simulink library "WECSim_Lib_Moorings"  (R2020b)
settings: Solver=VariableStepAuto  StartTime=0.0  StopTime=10.0  RelTol=1e-3
undefined symbols (not defined in the file or in its folder): mooring, simu, X, Y, Z
libraries: sm_lib x16, nesl_utility x6, $bdroot x6, WECSim_Lib_Body_Elements x3
settings Model: Creator=kmruehl  LastModifiedBy=jtgrasb

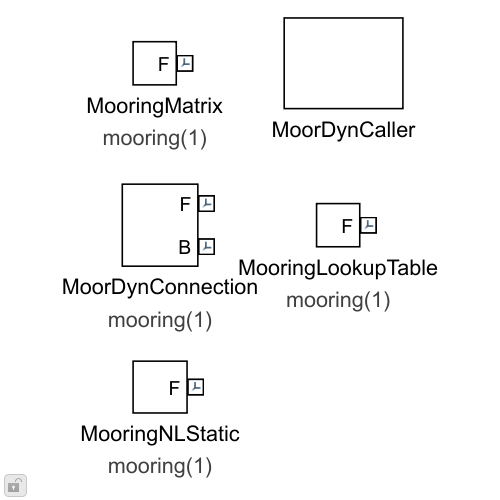
[thumbnail: Simulink's stored preview of the top-level diagram]
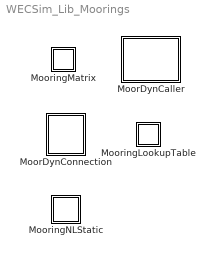
== system WECSim_Lib_Moorings ==
  MoorDynCaller : Subsystem  mask{simu=simu, mooring=mooring, InputFileText=Global Reference Frame option "Use Input File" is selected., numMoorDyn=0}
      mask prompts: simu "Simulation Class Name:"; mooring "Mooring Class Name:"; numMoorDyn "Number of MoorDyn Blocks"
      mask init:
      | if exist('mooring','var')
      |     h=[gcb '/Demux'];
      |     if str2num(get_param(h,'Outputs')) ~= simu.numMoorDyn
      |         % Delete old blocks
      |         fromBlocks = Simulink.findBlocks(gcb,'BlockType','From');
      |         gotoBlocks = Simulink.findBlocks(gcb,'BlockType','Goto');
      |         blocks = [fromBlocks;gotoBlocks];
      |         for ii=1:length(blocks)
      |             if ~contains(getfullname(blocks(ii)), 'Time')
      |                 line = get_param(blocks(ii),'LineHandles');
      |                 if line.Outport > 1
      |                     delete_line(line.Outport(1));
      |                 end
      |                 if line.Inport > 1
      |                     delete_line(line.Inport(1));
      |                 end
      |                 delete_block(blocks(ii))
      |             end
      |         end
      |         %% Set number of mux inputs and outputs
      |         h = [gcb '/muxDisp'];
      |         set_param(h,'Inputs',num2str(simu.numMoorDyn));
      |         h = [gcb '/muxVel'];
      |         set_param(h,'Inputs',num2str(simu.numMoorDyn));
      |         h = [gcb '/Demux'];
      |         set_param(h,'Outputs',num2str(simu.numMoorDyn));
      |         %% Add number of from and goto blocks according to MoorDyn connections
      |         for ii = 1:simu.numMoorDyn
      |             hDisp = add_block('simulink/Signal Routing/From',[gcb '/From'],'GotoTag',['moorDynDisp' num2str(ii)], 'MakeNameUnique', 'on');
      |             hVel = add_block('simulink/Signal Routing/From',[gcb '/From'],'GotoTag',['moorDynVel' num2str(ii)], 'MakeNameUnique', 'on');
      |             hForce = add_block('simulink/Signal Routing/Goto',[gcb '/Goto'],'GotoTag',['moorDynForce' num2str(ii)],'TagVisibility','global','MakeNameUnique', 'on');
      |             add_line(gcb,[get_param(hDisp,'Name') '/1'],[get_param([gcb '/muxDisp'],'Name') '/' num2str(ii)]);
      |             add_line(gcb,[get_param(hVel,'Name') '/1'],[get_param([gcb '/muxVel'],'Name') '/' num2str(ii)]);
      |             add_line(gcb,['Demux/' num2str(ii)],[get_param(hForce,'Name') '/1']);
      |         end
      |     end
      | end
      mask DialogControl InputFileGroup Prompt: Input File
      mask DialogControl CustomParameterGroup Prompt: Custom Parameters
      mask DialogControl mooringData Prompt: Mooring Data
      mask DialogControl simData Prompt: Simulation Data
  MoorDynConnection : Subsystem  mask(MoorDyn){mooring=mooring(1), InputFileText=Global Reference Frame option "Use Input File" is selected., MooringRef=0  0  0, moorDynLines=0}
      mask prompts: mooring "Mooring Name:"; MooringRef "Reference Location [m]:"; moorDynLines "Number of MoorDyn Lines:"
      mask help:
      | A mooring body that applies stiffness, damping and pretensions forces to the follower using a MoorDyn simulation. The response of the mooring body is relative to the global reference frame.
      |
      | The variable name input below must be 'mooring(i)' where i=1,2,...
      | mooring(i) must be defined in the input file with the following fields:
      |
      |     .name (required)
      |             String.
      |             Mooring name. Must comply with Matlab's variable naming rules.
      |     .location (optional)
      |             3x1 vector [x y z] in meters.
      |             Mooring location. Default = [0 0 0]
      |     .initial (optional)
      |             Struct
      |             Contains the initial position, angle and axis of the mooring body.
      |     .initial.displacement (optional)
      |             3x1 vector [x y z] in meters.
      |             Initial linear displacement from the ref position. Default = [0 0 0]
      |             This can can be set directly or with the setInitDisp() method.
      |     .initial.axis (optional)
      |             3x1 vector [x y z]
      |             Initial angular displacement axis. Default = [0 1 0]
      |             This can can be set directly or with the setInitDisp() method.
      |     .initial.angle (optional)
      |             Float.
      |             Initial angular displacement angle about axis in radians. Default = [0 0 0]
      |             This can can be set directly or with the setInitDisp() method.
      |     .moorDynLines (optional)
      |             Float.
      |             Number of lines for MoorDyn to use. Default = 0
      |     .moorDynNodes (optional)
      |             moorDynLines x 1 vector.
      |             Specifies the number of nodes per line in MoorDyn. Default = []
      mask init:
      | if exist('mooring','var')
      |     h=[gcb '/To Workspace'];
      |     responseName=['mooring' num2str(mooring.number) '_out'];
      |     set_param(h,'VariableName',responseName);
      |     % set from and goto block tags
      |     h=[gcb '/From'];
      |     set_param(h,'GotoTag',['moorDynForce' num2str(mooring.number)])
      |     h=[gcb '/Goto'];
      |     set_param(h,'GotoTag',['moorDynDisp' num2str(mooring.number)])
      |     h=[gcb '/Goto1'];
      |     set_param(h,'GotoTag',['moorDynVel' num2str(mooring.number)])
      | end
      settings: AttributesFormatString=%<mooring>
      mask Help:
      | A mooring body that applies stiffness, damping and pretensions forces to the follower using a MoorDyn simulation. The response of the mooring body is relative to the global reference frame.
      | 
      | The variable name input below must be 'mooring(i)' where i=1,2,...
      | mooring(i) must be defined in the input file with the following fields:
      | 
      |     .name (required)
      |             String.
      |             Mooring name. Must comply with Matlab's variable naming rules.
      |     .location (optional)
      |             3x1 vector [x y z] in meters.
      |             Mooring location. Default = [0 0 0]
      |     .initial (optional)
      |             Struct
      |             Contains the initial position, angle and axis of the mooring body.
      |     .initial.displacement (optional)
      |             3x1 vector [x y z] in meters.
      |             Initial linear displacement from the ref position. Default = [0 0 0]
      |             This can can be set directly or with the setInitDisp() method.
      |     .initial.axis (optional)
      |             3x1 vector [x y z]
      |             Initial angular displacement axis. Default = [0 1 0]
      |             This can can be set directly or with the setInitDisp() method.
      |     .initial.angle (optional)
      |             Float.
      |             Initial angular displacement angle about axis in radians. Default = [0 0 0]
      |             This can can be set directly or with the setInitDisp() method.
      |     .moorDynLines (optional)
      |             Float.
      |             Number of lines for MoorDyn to use. Default = 0
      |     .moorDynNodes (optional)
      |             moorDynLines x 1 vector.
      |             Specifies the number of nodes per line in MoorDyn. Default = []
      mask DialogControl InputFileGroup Prompt: Input File
      mask DialogControl CustomParameterGroup Prompt: Custom Parameters
      mask DialogControl mooringData Prompt: Mooring Data
  MooringLookupTable : Subsystem  mask{mooring=mooring(1)}
      mask prompts: mooring "Mooring Name:"
      mask init:
      | if exist('mooring','var')
      |     % toWorkSpace: outputs
      |     h=[gcb '/To Workspace'];
      |     responseName=['mooring' num2str(mooring.number) '_out'];
      |     set_param(h,'VariableName',responseName);
      | end
      settings: AttributesFormatString=%<mooring>
  MooringMatrix : Subsystem  mask(Mooring Matrix){mooring=mooring(1), InputFileText=Global Reference Frame option "Use Input File" is selected., loc=0 0 0, preTension=[0 0 0 0 0 0], stiffness={ '0', '0', '0', '0', '0', '0'; '0', '0', '0', '0', '0', '0'; '0', '0', '0', '0', '0', '0'; '0', '0', '0', '0', '0', '0'; '0', '0', '0', '0', '0', '0'; '0', '0', '0', '0', '0', '0' }, damping={ '0', '0', '0', '0', '0', '0'; '0', '0', '0', '0', '0', '0'; '0', '0', '0', '0', '0', '0'; '0', '0', '0', '0', '0', '0'; '0', '0', '0', '0', '0', '0'; '0', '0', '0', '0', '0', '0' }}
      mask prompts: mooring "Mooring Name:"; loc "Reference Location [m]:"; preTension "Pretension Force [N]:"; stiffness "Stiffness [N/m]:"; damping "Damping [N/m^2]:"
      mask help:
      | A mooring body that applies stiffness, damping and pretensions forces to the follower. The response of the mooring body is relative to the global reference frame.
      |
      | The variable name input below must be 'mooring(i)' where i=1,2,...
      | mooring(i) must be defined in the input file with the following fields:
      |
      |     .name (required)
      |             String.
      |             Mooring name. Must comply with Matlab's variable naming rules.
      |     .location (optional)
      |             3x1 vector [x y z] in meters.
      |             Mooring location. Default = [0 0 0]
      |     .initial (optional)
      |             Struct
      |             Contains the initial position, angle and axis of the mooring body.
      |     .initial.displacement (optional)
      |             3x1 vector [x y z] in meters.
      |             Initial linear displacement from the ref position. Default = [0 0 0]
      |             This can can be set directly or with the setInitDisp() method.
      |     .initial.axis (optional)
      |             3x1 vector [x y z]
      |             Initial angular displacement axis. Default = [0 1 0]
      |             This can can be set directly or with the setInitDisp() method.
      |     .initial.angle (optional)
      |             Float.
      |             Initial angular displacement angle about axis in radians. Default = [0 0 0]
      |             This can can be set directly or with the setInitDisp() method.
      |     .matrix (optional)
      |             Struct
      |             Contains the stiffness matrix, damping matrix and pretension of the mooring body.
      |     .matrix.stiffness (optional)
      |             6x6 vector.
      |             Mooring linear spring stiffness. Default = zeros(6)
      |     .matrix.damping (optional)
      |             6x6 vector.
      |             Mooring linear damping coefficient. Default = zeros(6)
      |     .matrix.preTension (optional)
      |             6x1 vector.
      |             Mooring preTension force. Default = [0 0 0 0 0 0]
      mask init:
      | if exist('mooring','var')
      |     % toWorkSpace: outputs
      |     h=[gcb '/To Workspace'];
      |     responseName=['mooring' num2str(mooring.number) '_out'];
      |     set_param(h,'VariableName',responseName);
      | end
      settings: AttributesFormatString=%<mooring>
      mask Help:
      | A mooring body that applies stiffness, damping and pretensions forces to the follower. The response of the mooring body is relative to the global reference frame.
      | 
      | The variable name input below must be 'mooring(i)' where i=1,2,...
      | mooring(i) must be defined in the input file with the following fields:
      | 
      |     .name (required)
      |             String.
      |             Mooring name. Must comply with Matlab's variable naming rules.
      |     .location (optional)
      |             3x1 vector [x y z] in meters.
      |             Mooring location. Default = [0 0 0]
      |     .initial (optional)
      |             Struct
      |             Contains the initial position, angle and axis of the mooring body.
      |     .initial.displacement (optional)
      |             3x1 vector [x y z] in meters.
      |             Initial linear displacement from the ref position. Default = [0 0 0]
      |             This can can be set directly or with the setInitDisp() method.
      |     .initial.axis (optional)
      |             3x1 vector [x y z]
      |             Initial angular displacement axis. Default = [0 1 0]
      |             This can can be set directly or with the setInitDisp() method.
      |     .initial.angle (optional)
      |             Float.
      |             Initial angular displacement angle about axis in radians. Default = [0 0 0]
      |             This can can be set directly or with the setInitDisp() method.
      |     .matrix (optional)
      |             Struct
      |             Contains the stiffness matrix, damping matrix and pretension of the mooring body.
      |     .matrix.stiffness (optional)
      |             6x6 vector.
      |             Mooring linear spring stiffness. Default = zeros(6)
      |     .matrix.damping (optional)
      |             6x6 vector.
      |             Mooring linear damping coefficient. Default = zeros(6)
      |     .matrix.preTension (optional)
      |             6x1 vector.
      |             Mooring preTension force. Default = [0 0 0 0 0 0]
      mask DialogControl InputFileGroup Prompt: Input File
      mask DialogControl CustomParameterGroup Prompt: Custom Parameters
      mask DialogControl matrix Prompt: Additional Parameters
  MooringNLStatic : Subsystem  mask(Mooring Matrix){mooring=mooring(1), nonlinearStaticData=mooring.nonlinearStaticData}
      mask prompts: mooring "Mooring Name:"; nonlinearStaticData "Mooring Data"
      mask help:
      | A mooring body that applies stiffness, damping and pretensions forces to the follower. The response of the mooring body is relative to the global reference frame.
      |
      | The variable name input below must be 'mooring(i)' where i=1,2,...
      | mooring(i) must be defined in the input file with the following fields:
      |
      |     .name (required)
      |             String.
      |             Mooring name. Must comply with Matlab's variable naming rules.
      |     .location (optional)
      |             3x1 vector [x y z] in meters.
      |             Mooring location. Default = [0 0 0]
      |     .initial (optional)
      |             Struct
      |             Contains the initial position, angle and axis of the mooring body.
      |     .initial.displacement (optional)
      |             3x1 vector [x y z] in meters.
      |             Initial linear displacement from the ref position. Default = [0 0 0]
      |             This can can be set directly or with the setInitDisp() method.
      |     .initial.axis (optional)
      |             3x1 vector [x y z]
      |             Initial angular displacement axis. Default = [0 1 0]
      |             This can can be set directly or with the setInitDisp() method.
      |     .initial.angle (optional)
      |             Float.
      |             Initial angular displacement angle about axis in radians. Default = [0 0 0]
      |             This can can be set directly or with the setInitDisp() method.
      |     .matrix (optional)
      |             Struct
      |             Contains the stiffness matrix, damping matrix and pretension of the mooring body.
      |     .matrix.stiffness (optional)
      |             6x6 vector.
      |             Mooring linear spring stiffness. Default = zeros(6)
      |     .matrix.damping (optional)
      |             6x6 vector.
      |             Mooring linear damping coefficient. Default = zeros(6)
      |     .matrix.preTension (optional)
      |             6x1 vector.
      |             Mooring preTension force. Default = [0 0 0 0 0 0]
      mask init:
      | if exist('mooring','var')
      |     % toWorkSpace: outputs
      |     h=[gcb '/To Workspace'];
      |     responseName=['mooring' num2str(mooring.number) '_out'];
      |     set_param(h,'VariableName',responseName);
      | end
      settings: AttributesFormatString=%<mooring>
      mask Help:
      | A mooring body that applies stiffness, damping and pretensions forces to the follower. The response of the mooring body is relative to the global reference frame.
      | 
      | The variable name input below must be 'mooring(i)' where i=1,2,...
      | mooring(i) must be defined in the input file with the following fields:
      | 
      |     .name (required)
      |             String.
      |             Mooring name. Must comply with Matlab's variable naming rules.
      |     .location (optional)
      |             3x1 vector [x y z] in meters.
      |             Mooring location. Default = [0 0 0]
      |     .initial (optional)
      |             Struct
      |             Contains the initial position, angle and axis of the mooring body.
      |     .initial.displacement (optional)
      |             3x1 vector [x y z] in meters.
      |             Initial linear displacement from the ref position. Default = [0 0 0]
      |             This can can be set directly or with the setInitDisp() method.
      |     .initial.axis (optional)
      |             3x1 vector [x y z]
      |             Initial angular displacement axis. Default = [0 1 0]
      |             This can can be set directly or with the setInitDisp() method.
      |     .initial.angle (optional)
      |             Float.
      |             Initial angular displacement angle about axis in radians. Default = [0 0 0]
      |             This can can be set directly or with the setInitDisp() method.
      |     .matrix (optional)
      |             Struct
      |             Contains the stiffness matrix, damping matrix and pretension of the mooring body.
      |     .matrix.stiffness (optional)
      |             6x6 vector.
      |             Mooring linear spring stiffness. Default = zeros(6)
      |     .matrix.damping (optional)
      |             6x6 vector.
      |             Mooring linear damping coefficient. Default = zeros(6)
      |     .matrix.preTension (optional)
      |             6x1 vector.
      |             Mooring preTension force. Default = [0 0 0 0 0 0]

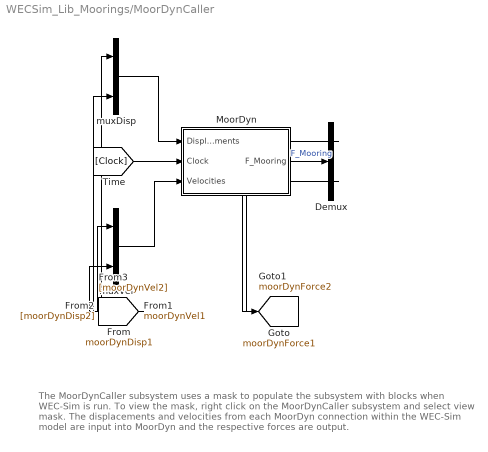
== system WECSim_Lib_Moorings/MoorDynCaller ==
  note: The MoorDynCaller subsystem uses a mask to populate the subsystem with blocks when WEC-Sim is run. To view the mask, right click on the MoorDynCaller subsystem and select view mask. The displacements and velocities from each MoorDyn connection within the WEC-Sim model are input into MoorDyn and the respective forces are output.
  Demux : Demux  Outputs=2
  MoorDyn : Subsystem  VariantControl=sv_moorDyn
  muxDisp : Mux  Inputs=2
  muxVel : Mux  Inputs=2
  tag scope: moorDynForce1=global, moorDynForce2=global
  wires:
  MoorDyn/1(F_Mooring) -> Demux/1  "F_Mooring"
  muxVel/1 -> MoorDyn/3(Velocities)
  muxDisp/1 -> MoorDyn/1(Displacements)
  [Clock] -> MoorDyn/2(Clock)
  [moorDynDisp1] -> muxDisp/1
  [moorDynVel1] -> muxVel/1
  Demux/1 -> [moorDynForce1]
  [moorDynDisp2] -> muxDisp/2
  [moorDynVel2] -> muxVel/2
  Demux/2 -> [moorDynForce2]

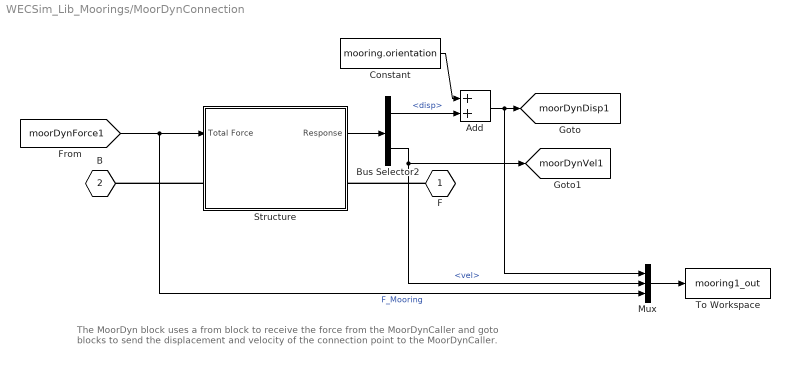
== system WECSim_Lib_Moorings/MoorDynConnection ==
  note: The MoorDyn block uses a from block to receive the force from the MoorDynCaller and goto blocks to send the displacement and velocity of the connection point to the MoorDynCaller.
  Add : Sum
  Bus Selector2 : BusSelector  OutputSignals=disp,vel
  Constant : Constant  Value=mooring.orientation
  Mux : Mux  Inputs=3
  Structure : Subsystem
  To Workspace : ToWorkspace  VariableName=mooring1_out  SaveFormat=Structure With Time  SampleTime=simu.dtOut
  F : PMIOPort  Side=Left
  B : PMIOPort  Port=2  Side=Left
  tag scope: moorDynDisp1=global, moorDynVel1=global
  wires:
  Add/1 -> [moorDynDisp1], Mux/1
  Constant/1 -> Add/1
  Bus Selector2/2 -> Mux/2, [moorDynVel1]  "<vel>"
  Mux/1 -> To Workspace/1
  Bus Selector2/1 -> Add/2  "<disp>"
  [moorDynForce1] -> Structure/1(Total Force), Mux/3  "F_Mooring"
  Structure/1(Response) -> Bus Selector2/1
  connections:
  F/RConn1 -- Structure/RConn1
  Structure/LConn1 -- B/RConn1

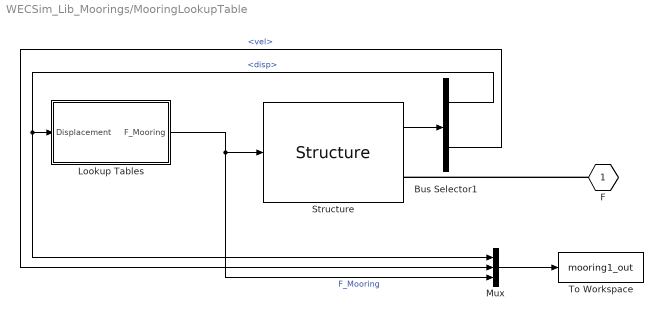
== system WECSim_Lib_Moorings/MooringLookupTable ==
  Bus Selector1 : BusSelector  OutputSignals=disp,vel
  Lookup Tables : Subsystem
  Mux : Mux  Inputs=3
  Structure : $bdroot/MooringMatrix/Structure  SystemSampleTime=-1  VariantActivationTime=update diagram  Latency=0  AutoFrameSizeCalculation=off
      link override Body Properties: GraphicType=None
  To Workspace : ToWorkspace  VariableName=mooring1_out  SaveFormat=Structure With Time  SampleTime=simu.dtOut
  F : PMIOPort  Side=Left
  wires:
  Mux/1 -> To Workspace/1
  Bus Selector1/2 -> Mux/2  "<vel>"
  Bus Selector1/1 -> Mux/1, Lookup Tables/1(Displacement)  "<disp>"
  Lookup Tables/1(F_Mooring) -> Mux/3, Structure/1  "F_Mooring"
  Structure/1 -> Bus Selector1/1
  connections:
  F/RConn1 -- Structure/RConn1

== system WECSim_Lib_Moorings/MooringMatrix ==
  Bus Selector2 : BusSelector  OutputSignals=disp,vel
  Mooring Matrix : Subsystem  VariantControl=sv_mooringMatrix
  Mux : Mux  Inputs=3
  Structure : Subsystem
  To Workspace : ToWorkspace  VariableName=mooring1_out  SaveFormat=Structure With Time  SampleTime=simu.dtOut
  F : PMIOPort  Side=Left
  wires:
  Structure/1(Response) -> Bus Selector2/1
  Mooring Matrix/1(F_Mooring) -> Mux/3, Structure/1(Total Force)  "F_Mooring"
  Bus Selector2/1 -> Mux/1, Mooring Matrix/1(Displacement)  "<disp>"
  Bus Selector2/2 -> Mux/2, Mooring Matrix/2(Velocity)  "<vel>"
  Mux/1 -> To Workspace/1
  connections:
  F/RConn1 -- Structure/RConn1

== system WECSim_Lib_Moorings/MooringNLStatic ==
  Bus Selector2 : BusSelector  OutputSignals=disp,vel
  Mooring Matrix : Subsystem  VariantControl=sv_mooringMatrix
  Mux : Mux  Inputs=3
  Structure : Subsystem
  To Workspace : ToWorkspace  VariableName=mooring1_out  SaveFormat=Structure With Time  SampleTime=simu.dtOut
  F : PMIOPort  Side=Left
  wires:
  Mux/1 -> To Workspace/1
  Bus Selector2/2 -> Mux/2  "<vel>"
  Bus Selector2/1 -> Mooring Matrix/1(Displacement), Mux/1  "<disp>"
  Mooring Matrix/1(F_Mooring) -> Structure/1(Total Force), Mux/3  "F_Mooring"
  Structure/1(Response) -> Bus Selector2/1
  connections:
  F/RConn1 -- Structure/RConn1

== system WECSim_Lib_Moorings/MoorDynCaller/MoorDyn ==
  Displacements : Inport
  Clock : Inport  Port=2
  Velocities : Inport  Port=3
  MoorDyn : Subsystem
  F_Mooring : Outport
  wires:
  MoorDyn/1(Flines) -> F_Mooring/1
  Clock/1 -> MoorDyn/2(Clock)
  Displacements/1 -> MoorDyn/3(Displacements)
  Velocities/1 -> MoorDyn/1(Velocities)

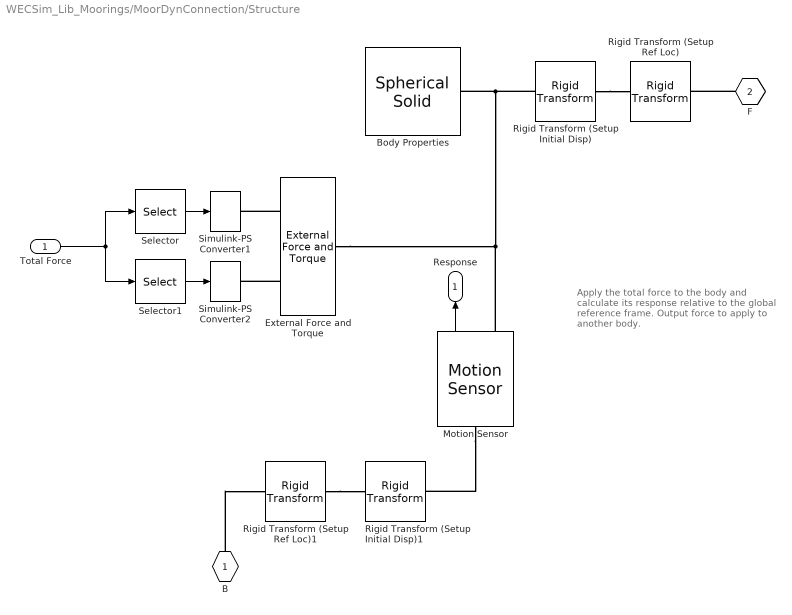
== system WECSim_Lib_Moorings/MoorDynConnection/Structure ==
  note: Apply the total force to the body and calculate its response relative to the global reference frame.
      |
      | Output force to apply to another body.
  Total Force : Inport
  Body Properties : sm_lib/Body Elements/Spherical Solid  GraphicAmbientColor=[0.15 0.15 0.15 1.0]  BasedOnType=Density  CenterOfMass=[0 0 0]  CenterOfMassUnits=m  GraphicDiffuseColor=[0 1 0]  Density=1000  DensityUnits=kg/(m^3)  DoExposeReferenceFrame=on  GraphicEmissiveColor=[0.0 0.0 0.0 1.0]  ExportEntireGeometry=off  SerializedExposedGeometries=<ExposedGeometries/>  SerializedFrames=<Frames/>  MarkerShape=Sphere  MarkerSize=10  GraphicType=None  InertiaType=Custom  Mass=0  MassUnits=kg  MomentsOfInertia=[0 0 0]  MomentsOfInertiaUnits=kg*m^2  GraphicOpacity=1  ProductsOfInertia=[0 0 0]  ProductsOfInertiaUnits=kg*m^2  GraphicShininess=75  GraphicSpecularColor=[0.5 0.5 0.5 1.0]  SphereRadius=1  SphereRadiusUnits=m  GraphicVisPropType=SimpleVisualProperties
  External Force and Torque : sm_lib/Forces and Torques/External Force and Torque  ForceResolutionFrame=World  EnableForceX=off  EnableForceY=off  EnableForceZ=off  EnableForce=on  TorqueResolutionFrame=World  EnableTorqueX=off  EnableTorqueY=off  EnableTorqueZ=off  EnableTorque=on
  Motion Sensor : WECSim_Lib_Body_Elements/Rigid Body/Hydrodynamic Body/Structure/Motion Sensor  SystemSampleTime=-1  VariantActivationTime=update diagram  Latency=0  AutoFrameSizeCalculation=off
  Rigid Transform (Setup Initial Disp) : sm_lib/Frames and Transforms/Rigid Transform  TranslationMethod=Cartesian  TranslationStandardOffset=0  TranslationStandardOffsetUnits=m  TranslationStandardAxis=+Z  TranslationCartesianOffset=mooring.initial.displacement  TranslationCartesianOffsetUnits=m  TranslationROffset=0  TranslationROffsetUnits=m  TranslationZOffset=0  TranslationZOffsetUnits=m  TranslationThetaOffset=0  TranslationThetaOffsetUnits=deg  RotationMethod=ArbitraryAxis  RotationAngleUnits=rad  RotationStandardAxis=+Y  RotationAngle=mooring.initial.angle  RotationArbitraryAxis=mooring.initial.axis  FollAlignAxisA=+X  BaseAlignAxisA=+Y  FollAlignAxisB=+Y  BaseAlignAxisB=+Z  RotationSequenceAxes=FollowerAxes  RotationSequence=XYX  RotationSequenceAngles=[0 0 0]  RotationSequenceAnglesUnits=deg  RotationMatrix=[1 0 0; 0 1 0; 0 0 1]  Quaternion=[1 0 0 0]
  Rigid Transform (Setup Initial Disp)1 : sm_lib/Frames and Transforms/Rigid Transform  TranslationMethod=Cartesian  TranslationStandardOffset=0  TranslationStandardOffsetUnits=m  TranslationStandardAxis=+Z  TranslationCartesianOffset=mooring.initial.displacement  TranslationCartesianOffsetUnits=m  TranslationROffset=0  TranslationROffsetUnits=m  TranslationZOffset=0  TranslationZOffsetUnits=m  TranslationThetaOffset=0  TranslationThetaOffsetUnits=deg  RotationMethod=ArbitraryAxis  RotationAngleUnits=rad  RotationStandardAxis=+Y  RotationAngle=mooring.initial.angle  RotationArbitraryAxis=mooring.initial.axis  FollAlignAxisA=+X  BaseAlignAxisA=+Y  FollAlignAxisB=+Y  BaseAlignAxisB=+Z  RotationSequenceAxes=FollowerAxes  RotationSequence=XYX  RotationSequenceAngles=[0 0 0]  RotationSequenceAnglesUnits=deg  RotationMatrix=[1 0 0; 0 1 0; 0 0 1]  Quaternion=[1 0 0 0]
  Rigid Transform (Setup Ref Loc) : sm_lib/Frames and Transforms/Rigid Transform  TranslationMethod=Cartesian  TranslationStandardOffset=0  TranslationStandardOffsetUnits=m  TranslationStandardAxis=+Z  TranslationCartesianOffset=mooring.location  TranslationCartesianOffsetUnits=m  TranslationROffset=0  TranslationROffsetUnits=m  TranslationZOffset=0  TranslationZOffsetUnits=m  TranslationThetaOffset=0  TranslationThetaOffsetUnits=deg  RotationMethod=None  RotationAngleUnits=rad  RotationStandardAxis=+Y  RotationAngle=0.05  RotationArbitraryAxis=[0.57735026918962584 0.57735026918962584 0.57735026918962584]  FollAlignAxisA=+X  BaseAlignAxisA=+Y  FollAlignAxisB=+Y  BaseAlignAxisB=+Z  RotationSequenceAxes=FollowerAxes  RotationSequence=XYX  RotationSequenceAngles=[0 0 0]  RotationSequenceAnglesUnits=deg  RotationMatrix=[1 0 0; 0 1 0; 0 0 1]  Quaternion=[1 0 0 0]
  Rigid Transform (Setup Ref Loc)1 : sm_lib/Frames and Transforms/Rigid Transform  TranslationMethod=Cartesian  TranslationStandardOffset=0  TranslationStandardOffsetUnits=m  TranslationStandardAxis=+Z  TranslationCartesianOffset=mooring.location  TranslationCartesianOffsetUnits=m  TranslationROffset=0  TranslationROffsetUnits=m  TranslationZOffset=0  TranslationZOffsetUnits=m  TranslationThetaOffset=0  TranslationThetaOffsetUnits=deg  RotationMethod=None  RotationAngleUnits=rad  RotationStandardAxis=+Y  RotationAngle=0.05  RotationArbitraryAxis=[0.57735026918962584 0.57735026918962584 0.57735026918962584]  FollAlignAxisA=+X  BaseAlignAxisA=+Y  FollAlignAxisB=+Y  BaseAlignAxisB=+Z  RotationSequenceAxes=FollowerAxes  RotationSequence=XYX  RotationSequenceAngles=[0 0 0]  RotationSequenceAnglesUnits=deg  RotationMatrix=[1 0 0; 0 1 0; 0 0 1]  Quaternion=[1 0 0 0]
  Selector : Selector  InputPortWidth=6  IndexOptions=Index vector (dialog)  Indices=[1:3]  OutputSizes=1
  Selector1 : Selector  InputPortWidth=6  IndexOptions=Index vector (dialog)  Indices=[4:6]  OutputSizes=1
  Simulink-PS Converter1 : nesl_utility/Simulink-PS Converter  PhysicalDomain=network_engine_domain  SubClassName=ps_input  LeftPortType=input  RightPortType=output  PseudoPeriodic=off  Frequencies=[]  NoiseDistribution=none  NoiseParameters=[]  Unit=1  AffineConversion=off  FilteringAndDerivatives=zero  SimscapeFilterOrder=1  InputFilterTimeConstant=0.001  UdotUserProvided=1
  Simulink-PS Converter2 : nesl_utility/Simulink-PS Converter  PhysicalDomain=network_engine_domain  SubClassName=ps_input  LeftPortType=input  RightPortType=output  PseudoPeriodic=off  Frequencies=[]  NoiseDistribution=none  NoiseParameters=[]  Unit=1  AffineConversion=off  FilteringAndDerivatives=zero  SimscapeFilterOrder=1  InputFilterTimeConstant=0.001  UdotUserProvided=1
  B : PMIOPort  Side=Left
  F : PMIOPort  Port=2  Side=Right
  Response : Outport
  wires:
  Total Force/1 -> Selector1/1, Selector/1
  Selector/1 -> Simulink-PS Converter1/1
  Selector1/1 -> Simulink-PS Converter2/1
  Motion Sensor/1 -> Response/1
  connections:
  Rigid Transform (Setup Ref Loc)1/RConn1 -- Rigid Transform (Setup Initial Disp)1/LConn1
  Motion Sensor/LConn1 -- Rigid Transform (Setup Initial Disp)1/RConn1
  External Force and Torque/LConn1 -- Simulink-PS Converter1/RConn1
  External Force and Torque/LConn2 -- Simulink-PS Converter2/RConn1
  Rigid Transform (Setup Initial Disp)/RConn1 -- Body Properties/RConn1 -- Motion Sensor/RConn1 -- External Force and Torque/RConn1
  F/RConn1 -- Rigid Transform (Setup Ref Loc)/LConn1
  Rigid Transform (Setup Initial Disp)/LConn1 -- Rigid Transform (Setup Ref Loc)/RConn1
  B/RConn1 -- Rigid Transform (Setup Ref Loc)1/LConn1

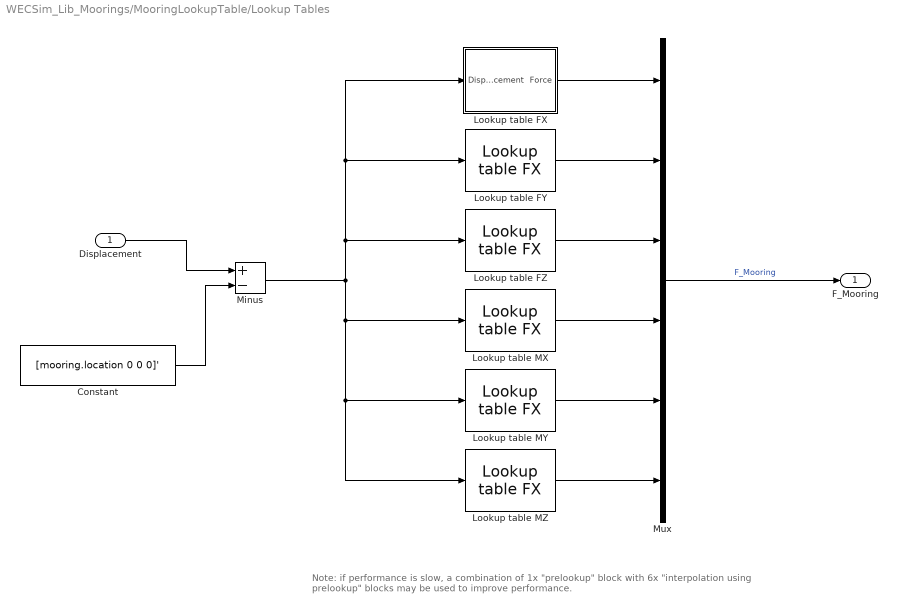
== system WECSim_Lib_Moorings/MooringLookupTable/Lookup Tables ==
  note: Note: if performance is slow, a combination of 1x "prelookup" block with 6x "interpolation using prelookup" blocks may be used to improve performance.
  Displacement : Inport
  Constant : Constant  Value=[mooring.location 0 0 0]'
  Lookup table FX : Subsystem  mask{forceComponent=mooring.lookupTable.FX}
      mask prompts: forceComponent "Force component:"
  Lookup table FY : $bdroot/MooringLookupTable/Lookup Tables/Lookup table FX  forceComponent=mooring.lookupTable.FY
  Lookup table FZ : $bdroot/MooringLookupTable/Lookup Tables/Lookup table FX  forceComponent=mooring.lookupTable.FZ
  Lookup table MX : $bdroot/MooringLookupTable/Lookup Tables/Lookup table FX  forceComponent=mooring.lookupTable.MX
  Lookup table MY : $bdroot/MooringLookupTable/Lookup Tables/Lookup table FX  forceComponent=mooring.lookupTable.MY
  Lookup table MZ : $bdroot/MooringLookupTable/Lookup Tables/Lookup table FX  forceComponent=mooring.lookupTable.MZ
  Minus : Sum  Inputs=+-
  Mux : Mux  Inputs=6
  F_Mooring : Outport
  wires:
  Minus/1 -> Lookup table MX/1, Lookup table MZ/1, Lookup table MY/1, Lookup table FY/1, Lookup table FX/1(Displacement), Lookup table FZ/1
  Lookup table MZ/1 -> Mux/6
  Lookup table MY/1 -> Mux/5
  Lookup table MX/1 -> Mux/4
  Lookup table FZ/1 -> Mux/3
  Lookup table FY/1 -> Mux/2
  Lookup table FX/1(Force) -> Mux/1
  Mux/1 -> F_Mooring/1  "F_Mooring"
  Displacement/1 -> Minus/1
  Constant/1 -> Minus/2

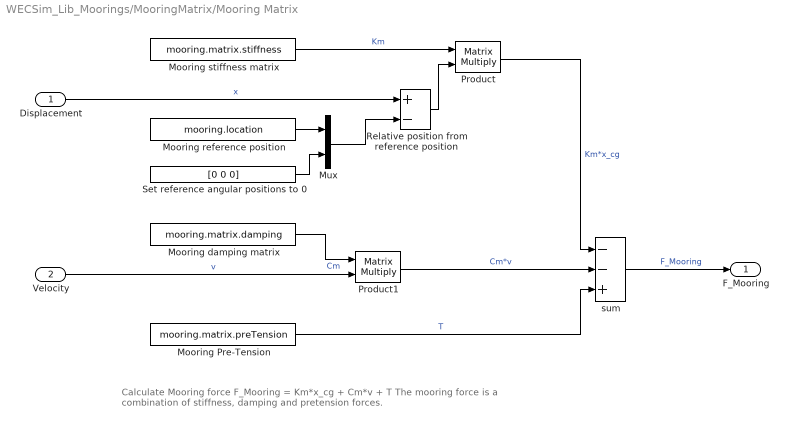
== system WECSim_Lib_Moorings/MooringMatrix/Mooring Matrix ==
  note: Calculate Mooring force
      |
      | F_Mooring = Km*x_cg + Cm*v + T
      | The mooring force is a combination of stiffness, damping and pretension forces.
  Displacement : Inport
  Velocity : Inport  Port=2
  Mooring Pre-Tension : Constant  Value=mooring.matrix.preTension
  Mooring damping matrix : Constant  Value=mooring.matrix.damping
  Mooring reference position : Constant  Value=mooring.location
  Mooring stiffness matrix : Constant  Value=mooring.matrix.stiffness
  Mux : Mux  Inputs=2
  Product : Product  Multiplication=Matrix(*)
  Product1 : Product  Multiplication=Matrix(*)
  Relative position from reference position : Sum  Inputs=+-
  Set reference angular positions to 0 : Constant  Value=[0 0 0]
  sum : Sum  Inputs=--+
  F_Mooring : Outport
  wires:
  Product/1 -> sum/1  "Km*x_cg"
  Product1/1 -> sum/2  "Cm*v"
  sum/1 -> F_Mooring/1  "F_Mooring"
  Mooring Pre-Tension/1 -> sum/3  "T"
  Mooring stiffness matrix/1 -> Product/1  "Km"
  Velocity/1 -> Product1/2  "v"
  Mooring damping matrix/1 -> Product1/1  "Cm"
  Displacement/1 -> Relative position from reference position/1  "x"
  Mooring reference position/1 -> Mux/1
  Set reference angular positions to 0/1 -> Mux/2
  Mux/1 -> Relative position from reference position/2
  Relative position from reference position/1 -> Product/2

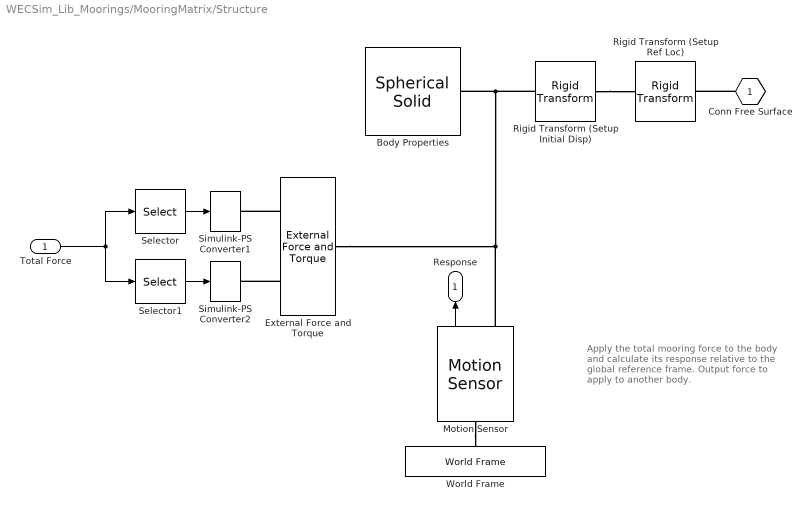
== system WECSim_Lib_Moorings/MooringMatrix/Structure ==
  note: Apply the total mooring force to the body and calculate its response relative to the global reference frame.
      |
      | Output force to apply to another body.
  Total Force : Inport
  Body Properties : sm_lib/Body Elements/Spherical Solid  GraphicAmbientColor=[0.15 0.15 0.15 1.0]  BasedOnType=Density  CenterOfMass=[0 0 0]  CenterOfMassUnits=m  GraphicDiffuseColor=[0.4 0.4 0.4]  Density=1000  DensityUnits=kg/(m^3)  DoExposeReferenceFrame=on  GraphicEmissiveColor=[0.0 0.0 0.0 1.0]  ExportEntireGeometry=off  SerializedExposedGeometries=<ExposedGeometries/>  SerializedFrames=<Frames/>  MarkerShape=Sphere  MarkerSize=10  GraphicType=Marker  InertiaType=Custom  Mass=0  MassUnits=kg  MomentsOfInertia=[0 0 0]  MomentsOfInertiaUnits=kg*m^2  GraphicOpacity=1  ProductsOfInertia=[0 0 0]  ProductsOfInertiaUnits=kg*m^2  GraphicShininess=75  GraphicSpecularColor=[0.5 0.5 0.5 1.0]  SphereRadius=5  SphereRadiusUnits=m  GraphicVisPropType=SimpleVisualProperties
  External Force and Torque : sm_lib/Forces and Torques/External Force and Torque  ForceResolutionFrame=World  EnableForceX=off  EnableForceY=off  EnableForceZ=off  EnableForce=on  TorqueResolutionFrame=World  EnableTorqueX=off  EnableTorqueY=off  EnableTorqueZ=off  EnableTorque=on
  Motion Sensor : WECSim_Lib_Body_Elements/Rigid Body/Hydrodynamic Body/Structure/Motion Sensor  SystemSampleTime=-1  VariantActivationTime=update diagram  Latency=0  AutoFrameSizeCalculation=off
  Rigid Transform (Setup Initial Disp) : sm_lib/Frames and Transforms/Rigid Transform  TranslationMethod=Cartesian  TranslationStandardOffset=0  TranslationStandardOffsetUnits=m  TranslationStandardAxis=+Z  TranslationCartesianOffset=mooring.initial.displacement  TranslationCartesianOffsetUnits=m  TranslationROffset=0  TranslationROffsetUnits=m  TranslationZOffset=0  TranslationZOffsetUnits=m  TranslationThetaOffset=0  TranslationThetaOffsetUnits=deg  RotationMethod=ArbitraryAxis  RotationAngleUnits=rad  RotationStandardAxis=+Y  RotationAngle=mooring.initial.angle  RotationArbitraryAxis=mooring.initial.axis  FollAlignAxisA=+X  BaseAlignAxisA=+Y  FollAlignAxisB=+Y  BaseAlignAxisB=+Z  RotationSequenceAxes=FollowerAxes  RotationSequence=XYX  RotationSequenceAngles=[0 0 0]  RotationSequenceAnglesUnits=deg  RotationMatrix=[1 0 0; 0 1 0; 0 0 1]  Quaternion=[1 0 0 0]
  Rigid Transform (Setup Ref Loc) : sm_lib/Frames and Transforms/Rigid Transform  TranslationMethod=Cartesian  TranslationStandardOffset=0  TranslationStandardOffsetUnits=m  TranslationStandardAxis=+Z  TranslationCartesianOffset=mooring.location  TranslationCartesianOffsetUnits=m  TranslationROffset=0  TranslationROffsetUnits=m  TranslationZOffset=0  TranslationZOffsetUnits=m  TranslationThetaOffset=0  TranslationThetaOffsetUnits=deg  RotationMethod=None  RotationAngleUnits=rad  RotationStandardAxis=+Y  RotationAngle=0.05  RotationArbitraryAxis=[0.57735026918962584 0.57735026918962584 0.57735026918962584]  FollAlignAxisA=+X  BaseAlignAxisA=+Y  FollAlignAxisB=+Y  BaseAlignAxisB=+Z  RotationSequenceAxes=FollowerAxes  RotationSequence=XYX  RotationSequenceAngles=[0 0 0]  RotationSequenceAnglesUnits=deg  RotationMatrix=[1 0 0; 0 1 0; 0 0 1]  Quaternion=[1 0 0 0]
  Selector : Selector  InputPortWidth=6  IndexOptions=Index vector (dialog)  Indices=[1:3]  OutputSizes=1
  Selector1 : Selector  InputPortWidth=6  IndexOptions=Index vector (dialog)  Indices=[4:6]  OutputSizes=1
  Simulink-PS Converter1 : nesl_utility/Simulink-PS Converter  PhysicalDomain=network_engine_domain  SubClassName=ps_input  LeftPortType=input  RightPortType=output  PseudoPeriodic=off  Frequencies=[]  NoiseDistribution=none  NoiseParameters=[]  Unit=1  AffineConversion=off  FilteringAndDerivatives=zero  SimscapeFilterOrder=1  InputFilterTimeConstant=0.001  UdotUserProvided=1
  Simulink-PS Converter2 : nesl_utility/Simulink-PS Converter  PhysicalDomain=network_engine_domain  SubClassName=ps_input  LeftPortType=input  RightPortType=output  PseudoPeriodic=off  Frequencies=[]  NoiseDistribution=none  NoiseParameters=[]  Unit=1  AffineConversion=off  FilteringAndDerivatives=zero  SimscapeFilterOrder=1  InputFilterTimeConstant=0.001  UdotUserProvided=1
  World Frame : sm_lib/Frames and Transforms/World Frame
  Conn Free Surface : PMIOPort  Side=Right
  Response : Outport
  wires:
  Total Force/1 -> Selector1/1, Selector/1
  Selector/1 -> Simulink-PS Converter1/1
  Selector1/1 -> Simulink-PS Converter2/1
  Motion Sensor/1 -> Response/1
  connections:
  External Force and Torque/LConn1 -- Simulink-PS Converter1/RConn1
  External Force and Torque/LConn2 -- Simulink-PS Converter2/RConn1
  Rigid Transform (Setup Initial Disp)/RConn1 -- Body Properties/RConn1 -- Motion Sensor/RConn1 -- External Force and Torque/RConn1
  Conn Free Surface/RConn1 -- Rigid Transform (Setup Ref Loc)/LConn1
  Rigid Transform (Setup Initial Disp)/LConn1 -- Rigid Transform (Setup Ref Loc)/RConn1
  Motion Sensor/LConn1 -- World Frame/RConn1

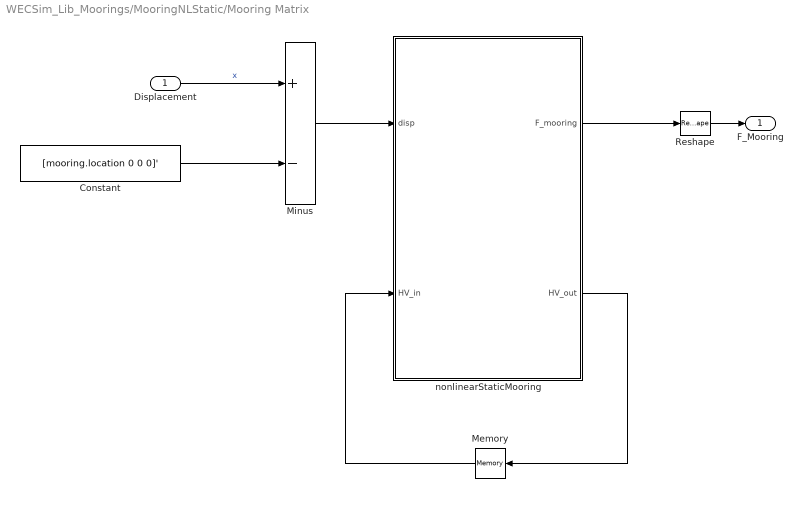
== system WECSim_Lib_Moorings/MooringNLStatic/Mooring Matrix ==
  Displacement : Inport
  Constant : Constant  Value=[mooring.location 0 0 0]'
  Memory : Memory  InitialCondition=nonlinearStaticData.HV0
  Minus : Sum  Inputs=+-
  Reshape : Reshape
  nonlinearStaticMooring : MATLAB Function  TreatAsAtomicUnit=on
  F_Mooring : Outport
  wires:
  Reshape/1 -> F_Mooring/1
  Displacement/1 -> Minus/1  "x"
  Constant/1 -> Minus/2
  nonlinearStaticMooring/1(F_mooring) -> Reshape/1
  nonlinearStaticMooring/2(HV_out) -> Memory/1
  Memory/1 -> nonlinearStaticMooring/2(HV_in)
  Minus/1 -> nonlinearStaticMooring/1(disp)

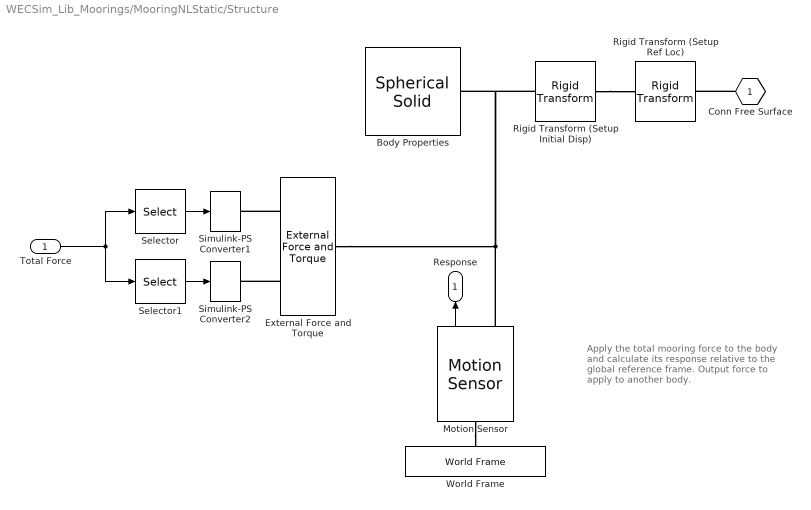
== system WECSim_Lib_Moorings/MooringNLStatic/Structure ==
  note: Apply the total mooring force to the body and calculate its response relative to the global reference frame.
      |
      | Output force to apply to another body.
  Total Force : Inport
  Body Properties : sm_lib/Body Elements/Spherical Solid  GraphicAmbientColor=[0.15 0.15 0.15 1.0]  BasedOnType=Density  CenterOfMass=[0 0 0]  CenterOfMassUnits=m  GraphicDiffuseColor=[0 1 0]  Density=1000  DensityUnits=kg/(m^3)  DoExposeReferenceFrame=on  GraphicEmissiveColor=[0.0 0.0 0.0 1.0]  ExportEntireGeometry=off  SerializedExposedGeometries=<ExposedGeometries/>  SerializedFrames=<Frames/>  MarkerShape=Sphere  MarkerSize=10  GraphicType=None  InertiaType=Custom  Mass=0  MassUnits=kg  MomentsOfInertia=[0 0 0]  MomentsOfInertiaUnits=kg*m^2  GraphicOpacity=1  ProductsOfInertia=[0 0 0]  ProductsOfInertiaUnits=kg*m^2  GraphicShininess=75  GraphicSpecularColor=[0.5 0.5 0.5 1.0]  SphereRadius=1  SphereRadiusUnits=m  GraphicVisPropType=SimpleVisualProperties
  External Force and Torque : sm_lib/Forces and Torques/External Force and Torque  ForceResolutionFrame=World  EnableForceX=off  EnableForceY=off  EnableForceZ=off  EnableForce=on  TorqueResolutionFrame=World  EnableTorqueX=off  EnableTorqueY=off  EnableTorqueZ=off  EnableTorque=on
  Motion Sensor : WECSim_Lib_Body_Elements/Rigid Body/Hydrodynamic Body/Structure/Motion Sensor  SystemSampleTime=-1  VariantActivationTime=update diagram  Latency=0  AutoFrameSizeCalculation=off
  Rigid Transform (Setup Initial Disp) : sm_lib/Frames and Transforms/Rigid Transform  TranslationMethod=Cartesian  TranslationStandardOffset=0  TranslationStandardOffsetUnits=m  TranslationStandardAxis=+Z  TranslationCartesianOffset=mooring.initial.displacement  TranslationCartesianOffsetUnits=m  TranslationROffset=0  TranslationROffsetUnits=m  TranslationZOffset=0  TranslationZOffsetUnits=m  TranslationThetaOffset=0  TranslationThetaOffsetUnits=deg  RotationMethod=ArbitraryAxis  RotationAngleUnits=rad  RotationStandardAxis=+Y  RotationAngle=mooring.initial.angle  RotationArbitraryAxis=mooring.initial.axis  FollAlignAxisA=+X  BaseAlignAxisA=+Y  FollAlignAxisB=+Y  BaseAlignAxisB=+Z  RotationSequenceAxes=FollowerAxes  RotationSequence=XYX  RotationSequenceAngles=[0 0 0]  RotationSequenceAnglesUnits=deg  RotationMatrix=[1 0 0; 0 1 0; 0 0 1]  Quaternion=[1 0 0 0]
  Rigid Transform (Setup Ref Loc) : sm_lib/Frames and Transforms/Rigid Transform  TranslationMethod=Cartesian  TranslationStandardOffset=0  TranslationStandardOffsetUnits=m  TranslationStandardAxis=+Z  TranslationCartesianOffset=mooring.location  TranslationCartesianOffsetUnits=m  TranslationROffset=0  TranslationROffsetUnits=m  TranslationZOffset=0  TranslationZOffsetUnits=m  TranslationThetaOffset=0  TranslationThetaOffsetUnits=deg  RotationMethod=None  RotationAngleUnits=rad  RotationStandardAxis=+Y  RotationAngle=0.05  RotationArbitraryAxis=[0.57735026918962584 0.57735026918962584 0.57735026918962584]  FollAlignAxisA=+X  BaseAlignAxisA=+Y  FollAlignAxisB=+Y  BaseAlignAxisB=+Z  RotationSequenceAxes=FollowerAxes  RotationSequence=XYX  RotationSequenceAngles=[0 0 0]  RotationSequenceAnglesUnits=deg  RotationMatrix=[1 0 0; 0 1 0; 0 0 1]  Quaternion=[1 0 0 0]
  Selector : Selector  InputPortWidth=6  IndexOptions=Index vector (dialog)  Indices=[1:3]  OutputSizes=1
  Selector1 : Selector  InputPortWidth=6  IndexOptions=Index vector (dialog)  Indices=[4:6]  OutputSizes=1
  Simulink-PS Converter1 : nesl_utility/Simulink-PS Converter  PhysicalDomain=network_engine_domain  SubClassName=ps_input  LeftPortType=input  RightPortType=output  PseudoPeriodic=off  Frequencies=[]  NoiseDistribution=none  NoiseParameters=[]  Unit=1  AffineConversion=off  FilteringAndDerivatives=zero  SimscapeFilterOrder=1  InputFilterTimeConstant=0.001  UdotUserProvided=1
  Simulink-PS Converter2 : nesl_utility/Simulink-PS Converter  PhysicalDomain=network_engine_domain  SubClassName=ps_input  LeftPortType=input  RightPortType=output  PseudoPeriodic=off  Frequencies=[]  NoiseDistribution=none  NoiseParameters=[]  Unit=1  AffineConversion=off  FilteringAndDerivatives=zero  SimscapeFilterOrder=1  InputFilterTimeConstant=0.001  UdotUserProvided=1
  World Frame : sm_lib/Frames and Transforms/World Frame
  Conn Free Surface : PMIOPort  Side=Right
  Response : Outport
  wires:
  Motion Sensor/1 -> Response/1
  Selector1/1 -> Simulink-PS Converter2/1
  Selector/1 -> Simulink-PS Converter1/1
  Total Force/1 -> Selector/1, Selector1/1
  connections:
  Motion Sensor/LConn1 -- World Frame/RConn1
  Rigid Transform (Setup Initial Disp)/LConn1 -- Rigid Transform (Setup Ref Loc)/RConn1
  Conn Free Surface/RConn1 -- Rigid Transform (Setup Ref Loc)/LConn1
  External Force and Torque/RConn1 -- Motion Sensor/RConn1 -- Body Properties/RConn1 -- Rigid Transform (Setup Initial Disp)/RConn1
  External Force and Torque/LConn2 -- Simulink-PS Converter2/RConn1
  External Force and Torque/LConn1 -- Simulink-PS Converter1/RConn1

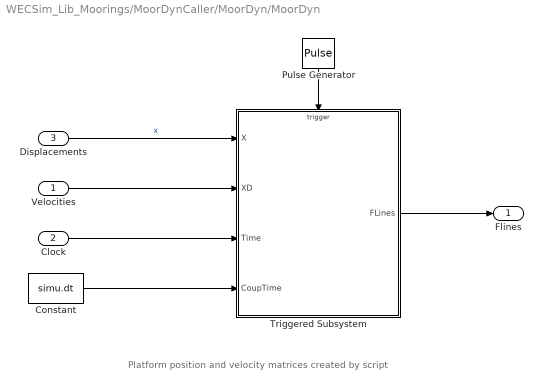
== system WECSim_Lib_Moorings/MoorDynCaller/MoorDyn/MoorDyn ==
  note: Platform position and velocity matrices created by script
  Velocities : Inport
  Clock : Inport  Port=2
  Displacements : Inport  Port=3
  Constant : Constant  Value=simu.dt
  Pulse Generator : DiscretePulseGenerator  PulseType=Time based  Amplitude=simu.endTime  Period=2*simu.dt  PulseWidth=50
  Triggered Subsystem : Subsystem  TreatAsAtomicUnit=on
  Flines : Outport
  wires:
  Displacements/1 -> Triggered Subsystem/1(X)  "x"
  Triggered Subsystem/1(FLines) -> Flines/1
  Clock/1 -> Triggered Subsystem/3(Time)
  Velocities/1 -> Triggered Subsystem/2(XD)
  Constant/1 -> Triggered Subsystem/4(CoupTime)
  Pulse Generator/1 -> Triggered Subsystem/Trigger

== system WECSim_Lib_Moorings/MooringLookupTable/Lookup Tables/Lookup table FX ==
  Displacement : Inport
  3-D Lookup Table3 : Lookup_n-D  NumberOfTableDimensions=6  BreakpointsForDimension1=mooring.lookupTable.X  BreakpointsForDimension2=mooring.lookupTable.Y  BreakpointsForDimension3=mooring.lookupTable.Z  BreakpointsForDimension4=mooring.lookupTable.RX  BreakpointsForDimension5=mooring.lookupTable.RY  BreakpointsForDimension6=mooring.lookupTable.RZ  Table=forceComponent  InternalRulePriority=Speed  RndMeth=Simplest  InputSameDT=on
      settings: InputPortMap=u0,u1,u2,u3,u4,u5
  Demux : Demux  Outputs=6
  Force : Outport
  wires:
  Displacement/1 -> Demux/1
  Demux/1 -> 3-D Lookup Table3/1
  Demux/6 -> 3-D Lookup Table3/6
  Demux/2 -> 3-D Lookup Table3/2
  Demux/4 -> 3-D Lookup Table3/4
  Demux/3 -> 3-D Lookup Table3/3
  Demux/5 -> 3-D Lookup Table3/5
  3-D Lookup Table3/1 -> Force/1

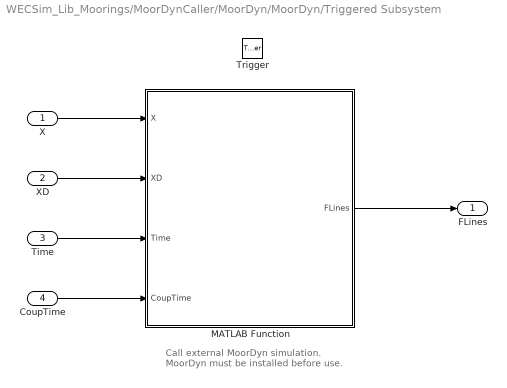
== system WECSim_Lib_Moorings/MoorDynCaller/MoorDyn/MoorDyn/Triggered Subsystem ==
  note: Call external MoorDyn simulation. MoorDyn must be installed before use.
  X : Inport
  XD : Inport  Port=2
  Time : Inport  Port=3
  CoupTime : Inport  Port=4
  Trigger : TriggerPort  TriggerType=either  VariantControl=(inherit)
  MATLAB Function : MATLAB Function  TreatAsAtomicUnit=on
  FLines : Outport
  wires:
  CoupTime/1 -> MATLAB Function/4(CoupTime)
  Time/1 -> MATLAB Function/3(Time)
  XD/1 -> MATLAB Function/2(XD)
  MATLAB Function/1(FLines) -> FLines/1
  X/1 -> MATLAB Function/1(X)

== matlab function WECSim_Lib_Moorings/MoorDynCaller/MoorDyn/MoorDyn/Triggered Subsystem/MATLAB Function ==
  data: X input; FLines output; XD input; Time input; CoupTime input
function FLines  = MoorDyn_matlab_FCN(X,XD,Time,CoupTime)

FLines = zeros(1,length(X));
FLines  = MoorDyn_matlab_FCN(X,XD,Time,CoupTime);

end

== matlab function WECSim_Lib_Moorings/MooringNLStatic/Mooring Matrix/nonlinearStaticMooring ==
  data: disp input size=[6 1]; F_mooring output size=[6 1]; HV_in input size=size(nonlinearStaticData.HV0); HV_out output size=size(nonlinearStaticData.HV0); nonlinearStaticData parameter
function [F_mooring, HV_out] = nlsMooring(disp, HV_in, nonlinearStaticData)

F_mooring = zeros(6, 1);
HV_out = zeros(nonlinearStaticData.nLines, 2);
[F_mooring, HV_out] = nonLinearStaticMooring(disp, HV_in, nonlinearStaticData);

end
